simulink library "WECSim_Lib_PTOSim"  (R2020b)
settings: Solver=ode45  StartTime=0.0  StopTime=10.0  RelTol=1e-3  EnableMultiTasking=on
undefined symbols (not defined in the file or in its folder): DiscIntNeverNeededParam, magnitude, ptoSim, simu
libraries: $bdroot x3, simulink x2
(part 2 of 2)

== system WECSim_Lib_PTOSim/Hydraulic/Compressible Fluid Piston/dPa_dt ==
  Pos : Inport
  Vel : Inport  Port=2
  QA : Inport  Port=3
  Add : Sum
  Add1 : Sum  Inputs=+-
  Constant : Constant  Value=ptoSim.hydPistonCompressible.Ap_A
  Constant1 : Constant  Value=ptoSim.hydPistonCompressible.bulkModulus
  Constant2 : Constant  Value=ptoSim.hydPistonCompressible.xi_piston
  Constant3 : Constant  Value=ptoSim.hydPistonCompressible.Ap_A
  Divide : Product  Inputs=/*
  Divide1 : Product  Inputs=*/
  Product : Product
  Product1 : Product
  Saturation : Saturate  UpperLimit=inf  LowerLimit=1e-10
  dPA_dt : Outport
  wires:
  Divide1/1 -> Product1/1
  Constant3/1 -> Divide1/2
  Constant1/1 -> Divide1/1
  Saturation/1 -> Divide/1
  Vel/1 -> Product/1
  Product1/1 -> Divide/2
  Divide/1 -> dPA_dt/1
  Add/1 -> Product1/2
  Constant/1 -> Product/2
  QA/1 -> Add/2
  Product/1 -> Add/1
  Pos/1 -> Add1/2
  Constant2/1 -> Add1/1
  Add1/1 -> Saturation/1

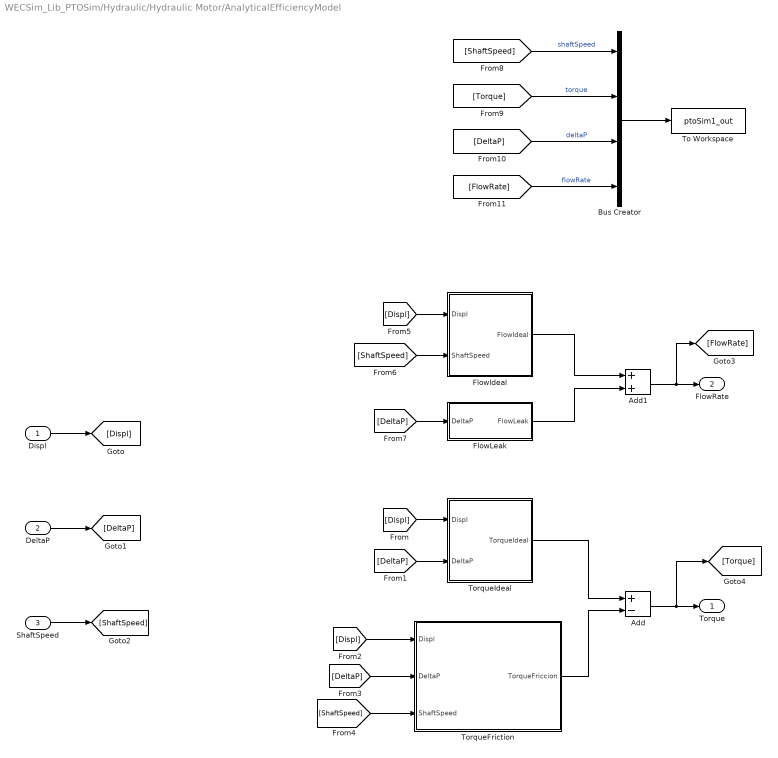
== system WECSim_Lib_PTOSim/Hydraulic/Hydraulic Motor/AnalyticalEfficiencyModel ==
  Displ : Inport
  DeltaP : Inport  Port=2
  ShaftSpeed : Inport  Port=3
  Add : Sum  Inputs=+-
  Add1 : Sum
  Bus Creator : BusCreator  Inputs=4
  FlowIdeal : Subsystem
  FlowLeak : Subsystem
  To Workspace : ToWorkspace  VariableName=ptoSim1_out  SaveFormat=Structure With Time  SampleTime=-1
  TorqueFriction : Subsystem
  TorqueIdeal : Subsystem
  Torque : Outport
  FlowRate : Outport  Port=2
  wires:
  Bus Creator/1 -> To Workspace/1
  Add/1 -> [Torque], Torque/1
  TorqueIdeal/1(TorqueIdeal) -> Add/1
  TorqueFriction/1(TorqueFriccion) -> Add/2
  Displ/1 -> [Displ]
  DeltaP/1 -> [DeltaP]
  ShaftSpeed/1 -> [ShaftSpeed]
  [Displ] -> TorqueIdeal/1(Displ)
  [DeltaP] -> TorqueIdeal/2(DeltaP)
  [DeltaP] -> TorqueFriction/2(DeltaP)
  [Displ] -> TorqueFriction/1(Displ)
  [ShaftSpeed] -> TorqueFriction/3(ShaftSpeed)
  FlowIdeal/1(FlowIdeal) -> Add1/1
  FlowLeak/1(FlowLeak) -> Add1/2
  Add1/1 -> [FlowRate], FlowRate/1
  [Displ] -> FlowIdeal/1(Displ)
  [ShaftSpeed] -> FlowIdeal/2(ShaftSpeed)
  [DeltaP] -> FlowLeak/1(DeltaP)
  [ShaftSpeed] -> Bus Creator/1  "shaftSpeed"
  [Torque] -> Bus Creator/2  "torque"
  [DeltaP] -> Bus Creator/3  "deltaP"
  [FlowRate] -> Bus Creator/4  "flowRate"

== system WECSim_Lib_PTOSim/Hydraulic/Hydraulic Motor/TabulatedEfficiency ==
  Displ : Inport
  DeltaP : Inport  Port=2
  ShaftSpeed : Inport  Port=3
  Bus Creator : BusCreator  Inputs=4
  Constant : Constant  Value=ptoSim.hydraulicMotor.displacement
  Constant2 : Constant  Value=ptoSim.hydraulicMotor.displacement
  Divide : Product  Inputs=/*
  Gain : Gain  Gain=1/((100^3)*(2*pi))
  Gain1 : Gain  Gain=1/((100^3)*(2*pi))
  Gain2 : Gain  Gain=2*pi/60
  MechanicalEfficiency : Lookup_n-D  BreakpointsForDimension1=ptoSim.hydraulicMotor.effTableShaftSpeed  BreakpointsForDimension2=ptoSim.hydraulicMotor.effTableDeltaP  Table=ptoSim.hydraulicMotor.effTableMechEff  InternalRulePriority=Speed  RndMeth=Simplest  InputSameDT=on
      settings: InputPortMap=u0,u1
  Product : Product
  Product1 : Product  Inputs=3
  Product2 : Product
  Product4 : Product
  To Workspace : ToWorkspace  VariableName=ptoSim1_out  SaveFormat=Structure With Time  SampleTime=-1
  VolumetricEfficiency : Lookup_n-D  BreakpointsForDimension1=ptoSim.hydraulicMotor.effTableShaftSpeed  BreakpointsForDimension2=ptoSim.hydraulicMotor.effTableDeltaP  Table=ptoSim.hydraulicMotor.effTableVolEff  InternalRulePriority=Speed  RndMeth=Simplest  InputSameDT=on
      settings: InputPortMap=u0,u1
  Torque : Outport
  FlowRate : Outport  Port=2
  wires:
  ShaftSpeed/1 -> MechanicalEfficiency/2, Gain2/1, VolumetricEfficiency/2, Bus Creator/1  "shaftSpeed"
  Divide/1 -> Bus Creator/4, FlowRate/1  "flowRate"
  Product1/1 -> Bus Creator/2, Torque/1  "torque"
  Gain1/1 -> Product/2
  Product/1 -> Divide/2
  Gain/1 -> Product1/1
  VolumetricEfficiency/1 -> Divide/1
  DeltaP/1 -> Product1/2, VolumetricEfficiency/1, MechanicalEfficiency/1, Bus Creator/3  "deltaP"
  MechanicalEfficiency/1 -> Product1/3
  Product2/1 -> Gain1/1
  Bus Creator/1 -> To Workspace/1
  Product4/1 -> Gain/1
  Constant/1 -> Product2/2
  Displ/1 -> Product4/2, Product2/1
  Constant2/1 -> Product4/1
  Gain2/1 -> Product/1

== system WECSim_Lib_PTOSim/Hydraulic/Rectifying Check Valve/Valve1 ==
  DeltaP : Inport
  Av : Subsystem
  Constant : Constant  Value=ptoSim.rectifyingCheckValve.rho
  Divide : Product  Inputs=/*
  Gain : Gain  Gain=ptoSim.rectifyingCheckValve.k1
  Gain1 : Gain  Gain=2
  Gain2 : Gain  Gain=ptoSim.rectifyingCheckValve.Cd
  Product : Product
  Product1 : Product
  Sqrt : Sqrt  SaturateOnIntegerOverflow=on
  Trigonometric Function : Trigonometry  Operator=tanh
  Qcv : Outport
  wires:
  DeltaP/1 -> Gain/1, Gain1/1, Av/1(DeltaP)
  Gain/1 -> Trigonometric Function/1
  Trigonometric Function/1 -> Product/1
  Gain1/1 -> Product/2
  Product/1 -> Divide/2
  Constant/1 -> Divide/1
  Divide/1 -> Sqrt/1
  Sqrt/1 -> Gain2/1
  Gain2/1 -> Product1/1
  Av/1(Av) -> Product1/2
  Product1/1 -> Qcv/1

== system WECSim_Lib_PTOSim/Motion Conversion/Rotary to Linear Adjustable Rod/Angle Calculation for PTO ==
  angPos : Inport
  Add : Sum  Inputs=+-
  Add1 : Sum  Inputs=+-
  Constant1 : Constant  Value=ptoSim.adjustableRod.crank
  Constant2 : Constant  Value=ptoSim.adjustableRod.crank
  Constant3 : Constant  Value=ptoSim.adjustableRod.offset
  Distance btw flap joint & rod joint along x-axis : Subsystem  AncestorBlock=|
      | PTOSim_Lib/Motion Conversion/Rotary to Linear
      | Adjustable Rod/Angular to Linear
      | Velocity/Subsystem/Distance btw flap joint & rod joint
      | along x-axis
  Divide : Product  Inputs=*/
  Divide1 : Product  Inputs=*/
  Product : Product
  Product1 : Product
  Subsystem1 : Subsystem  AncestorBlock=|
      | PTOSim_Lib/Motion Conversion/Rotary to Linear
      | Adjustable Rod/Angular to Linear
      | Velocity/Subsystem
  Subsystem2 : Subsystem  AncestorBlock=|
      | PTOSim_Lib/Motion Conversion/Rotary to Linear
      | Adjustable Rod/Angular to Linear
      | Velocity/Subsystem
  Trigonometric Function : Trigonometry
  Trigonometric Function1 : Trigonometry  Operator=cos
  Cos_gamma : Outport
  Sin_gamma : Outport  Port=2
  wires:
  Trigonometric Function/1 -> Product/1
  Product/1 -> Add/1
  Distance btw flap joint & rod joint along x-axis/1(d) -> Add/2
  Constant2/1 -> Product/2
  Add/1 -> Divide/1
  Subsystem1/1(rodLength) -> Divide/2
  Divide/1 -> Cos_gamma/1
  Subsystem2/1(rodLength) -> Divide1/2
  Trigonometric Function1/1 -> Product1/1
  Constant1/1 -> Product1/2
  Product1/1 -> Add1/1
  Constant3/1 -> Add1/2
  Add1/1 -> Divide1/1
  angPos/1 -> Subsystem1/1(angPos), Subsystem2/1(angPos), Trigonometric Function1/1, Trigonometric Function/1
  Divide1/1 -> Sin_gamma/1

== system WECSim_Lib_PTOSim/Motion Conversion/Rotary to Linear Adjustable Rod/Angular to Linear Position ==
  angPos : Inport
  Add1 : Sum  Inputs=-+
  Add2 : Sum  Inputs=+-
  Add5 : Sum
  Add6 : Sum  Inputs=+-
  Constant1 : Constant  Value=ptoSim.adjustableRod.rodInit
  Constant2 : Constant  Value=ptoSim.adjustableRod.crank
  Constant3 : Constant  Value=ptoSim.adjustableRod.offset
  Constant7 : Constant  Value=ptoSim.adjustableRod.crank
  Distance btw flap joint & rod joint along x-axis : Subsystem
  Math Function1 : Math  Operator=square  SignedPower=on  SaturateOnIntegerOverflow=on
  Math Function6 : Math  Operator=square  SignedPower=on  SaturateOnIntegerOverflow=on
  Product1 : Product  Inputs=**
  Product7 : Product  Inputs=**
  Sqrt2 : Sqrt  SaturateOnIntegerOverflow=on
  Trigonometric Function1 : Trigonometry  Operator=cos
  Trigonometric Function5 : Trigonometry
  linearPos : Outport
  wires:
  angPos/1 -> Trigonometric Function5/1, Trigonometric Function1/1
  Add1/1 -> linearPos/1
  Add2/1 -> Math Function1/1
  Trigonometric Function5/1 -> Product7/2
  Product7/1 -> Add6/2
  Add6/1 -> Math Function6/1
  Math Function6/1 -> Add5/2
  Add5/1 -> Sqrt2/1
  Sqrt2/1 -> Add1/2
  Constant1/1 -> Add1/1
  Constant2/1 -> Product1/1
  Trigonometric Function1/1 -> Product1/2
  Product1/1 -> Add2/1
  Constant3/1 -> Add2/2
  Math Function1/1 -> Add5/1
  Constant7/1 -> Product7/1
  Distance btw flap joint & rod joint along x-axis/1(d) -> Add6/1

== system WECSim_Lib_PTOSim/Motion Conversion/Rotary to Linear Adjustable Rod/Angular to Linear Velocity ==
  angPos : Inport
  angVel : Inport  Port=2
  Add1 : Sum  Inputs=+-
  Add2 : Sum  Inputs=+-
  Add3 : Sum  Inputs=-+
  Constant1 : Constant  Value=ptoSim.adjustableRod.crank
  Constant2 : Constant  Value=ptoSim.adjustableRod.crank
  Constant3 : Constant  Value=ptoSim.adjustableRod.offset
  Constant7 : Constant  Value=ptoSim.adjustableRod.crank
  Distance btw flap joint & rod joint along x-axis : Subsystem
  Divide1 : Product  Inputs=*/
  Product1 : Product  Inputs=**
  Product2 : Product  Inputs=***
  Product3 : Product  Inputs=**
  Product4 : Product  Inputs=***
  Product7 : Product  Inputs=**
  Subsystem : Subsystem
  Trigonometric Function1 : Trigonometry  Operator=cos
  Trigonometric Function2 : Trigonometry  Operator=cos
  Trigonometric Function5 : Trigonometry
  linearVel : Outport
  wires:
  Add2/1 -> Product2/1
  Constant2/1 -> Product1/1
  Trigonometric Function1/1 -> Product1/2
  Product1/1 -> Add2/1
  Constant3/1 -> Add2/2
  Trigonometric Function5/1 -> Product7/2
  Product7/1 -> Add1/1, Product2/2
  Constant7/1 -> Product7/1
  angVel/1 -> Product2/3, Product4/1
  Distance btw flap joint & rod joint along x-axis/1(d) -> Add1/2
  Constant1/1 -> Product3/1
  Trigonometric Function2/1 -> Product3/2
  Product3/1 -> Product4/3
  angPos/1 -> Trigonometric Function5/1, Trigonometric Function2/1, Trigonometric Function1/1, Subsystem/1(angPos)
  Add1/1 -> Product4/2
  Subsystem/1(rodLength) -> Divide1/2
  Product2/1 -> Add3/1
  Product4/1 -> Add3/2
  Add3/1 -> Divide1/1
  Divide1/1 -> linearVel/1

== system WECSim_Lib_PTOSim/Motion Conversion/Rotary to Linear Crank/Angular to Linear Position ==
  angPos : Inport
  Add1 : Sum  Inputs=++-
  Add2 : Sum  Inputs=+-
  Add5 : Sum  Inputs=+-
  Constant1 : Constant  Value=ptoSim.linearCrank.rodLength
  Constant2 : Constant  Value=ptoSim.linearCrank.crank
  Constant3 : Constant  Value=ptoSim.linearCrank.offset
  Constant7 : Constant  Value=ptoSim.linearCrank.crank
  Initial Distance btw flap joint & crank joint along x-axis : Subsystem
  Math Function1 : Math  Operator=square  SignedPower=on  SaturateOnIntegerOverflow=on
  Math Function2 : Math  Operator=square  SignedPower=on  SaturateOnIntegerOverflow=on
  Product1 : Product  Inputs=**
  Product7 : Product  Inputs=**
  Sqrt2 : Sqrt  SaturateOnIntegerOverflow=on
  Trigonometric Function1 : Trigonometry  Operator=cos
  Trigonometric Function5 : Trigonometry
  linearPos : Outport
  wires:
  angPos/1 -> Trigonometric Function1/1, Trigonometric Function5/1
  Add2/1 -> Math Function1/1
  Trigonometric Function5/1 -> Product7/2
  Add5/1 -> Sqrt2/1
  Constant2/1 -> Product1/1
  Trigonometric Function1/1 -> Product1/2
  Product1/1 -> Add2/1
  Constant3/1 -> Add2/2
  Constant7/1 -> Product7/1
  Initial Distance btw flap joint & crank joint along x-axis/1(d) -> Add1/3
  Constant1/1 -> Math Function2/1
  Math Function1/1 -> Add5/2
  Sqrt2/1 -> Add1/2
  Product7/1 -> Add1/1
  Add1/1 -> linearPos/1
  Math Function2/1 -> Add5/1

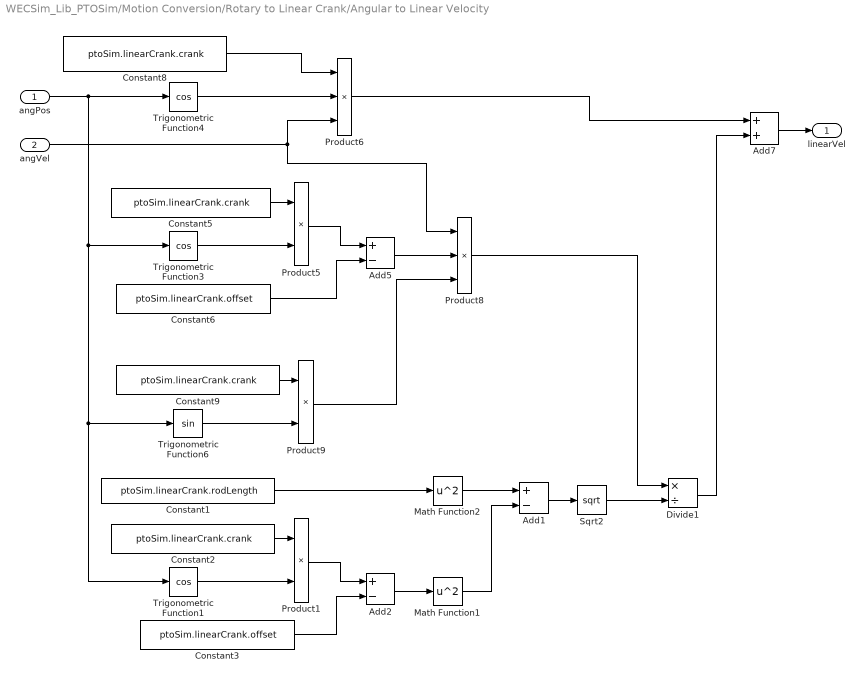
== system WECSim_Lib_PTOSim/Motion Conversion/Rotary to Linear Crank/Angular to Linear Velocity ==
  angPos : Inport
  angVel : Inport  Port=2
  Add1 : Sum  Inputs=+-
  Add2 : Sum  Inputs=+-
  Add5 : Sum  Inputs=+-
  Add7 : Sum
  Constant1 : Constant  Value=ptoSim.linearCrank.rodLength
  Constant{2,5,8..9} (4 alike) : Constant  Value=ptoSim.linearCrank.crank
  Constant3 : Constant  Value=ptoSim.linearCrank.offset
  Constant6 : Constant  Value=ptoSim.linearCrank.offset
  Divide1 : Product  Inputs=*/
  Math Function1 : Math  Operator=square  SignedPower=on  SaturateOnIntegerOverflow=on
  Math Function2 : Math  Operator=square  SignedPower=on  SaturateOnIntegerOverflow=on
  Product1 : Product  Inputs=**
  Product5 : Product  Inputs=**
  Product6 : Product  Inputs=***
  Product8 : Product  Inputs=***
  Product9 : Product  Inputs=**
  Sqrt2 : Sqrt  SaturateOnIntegerOverflow=on
  Trigonometric Function1 : Trigonometry  Operator=cos
  Trigonometric Function3 : Trigonometry  Operator=cos
  Trigonometric Function4 : Trigonometry  Operator=cos
  Trigonometric Function6 : Trigonometry
  linearVel : Outport
  wires:
  Add7/1 -> linearVel/1
  Trigonometric Function4/1 -> Product6/2
  Constant8/1 -> Product6/1
  Product6/1 -> Add7/1
  Constant5/1 -> Product5/1
  Trigonometric Function3/1 -> Product5/2
  Product5/1 -> Add5/1
  Constant6/1 -> Add5/2
  Constant9/1 -> Product9/1
  Trigonometric Function6/1 -> Product9/2
  angVel/1 -> Product8/1, Product6/3
  Add5/1 -> Product8/2
  Product9/1 -> Product8/3
  angPos/1 -> Trigonometric Function1/1, Trigonometric Function6/1, Trigonometric Function3/1, Trigonometric Function4/1
  Add2/1 -> Math Function1/1
  Add1/1 -> Sqrt2/1
  Constant2/1 -> Product1/1
  Trigonometric Function1/1 -> Product1/2
  Product1/1 -> Add2/1
  Constant3/1 -> Add2/2
  Constant1/1 -> Math Function2/1
  Math Function1/1 -> Add1/2
  Sqrt2/1 -> Divide1/2
  Product8/1 -> Divide1/1
  Divide1/1 -> Add7/2
  Math Function2/1 -> Add1/1

== system WECSim_Lib_PTOSim/Motion Conversion/Rotary to Linear Crank/Subsystem ==
  angle : Inport
  Add : Sum  Inputs=+-
  Add1 : Sum  Inputs=+-
  Constant : Constant
  Constant2 : Constant  Value=ptoSim.linearCrank.crank
  Constant3 : Constant  Value=ptoSim.linearCrank.offset
  Constant4 : Constant  Value=ptoSim.linearCrank.rodLength
  Divide : Product  Inputs=*/
  Product : Product
  Sqrt : Sqrt  SaturateOnIntegerOverflow=on
  Square : Math  Operator=square  SignedPower=on  SaturateOnIntegerOverflow=on
  Trigonometric Function : Trigonometry  Operator=cos
  abs(cos_gamma) : Outport
  wires:
  angle/1 -> Trigonometric Function/1
  Trigonometric Function/1 -> Product/1
  Constant2/1 -> Product/2
  Product/1 -> Add/1
  Constant3/1 -> Add/2
  Add/1 -> Divide/1
  Constant4/1 -> Divide/2
  Divide/1 -> Square/1
  Square/1 -> Add1/2
  Add1/1 -> Sqrt/1
  Constant/1 -> Add1/1
  Sqrt/1 -> abs(cos_gamma)/1

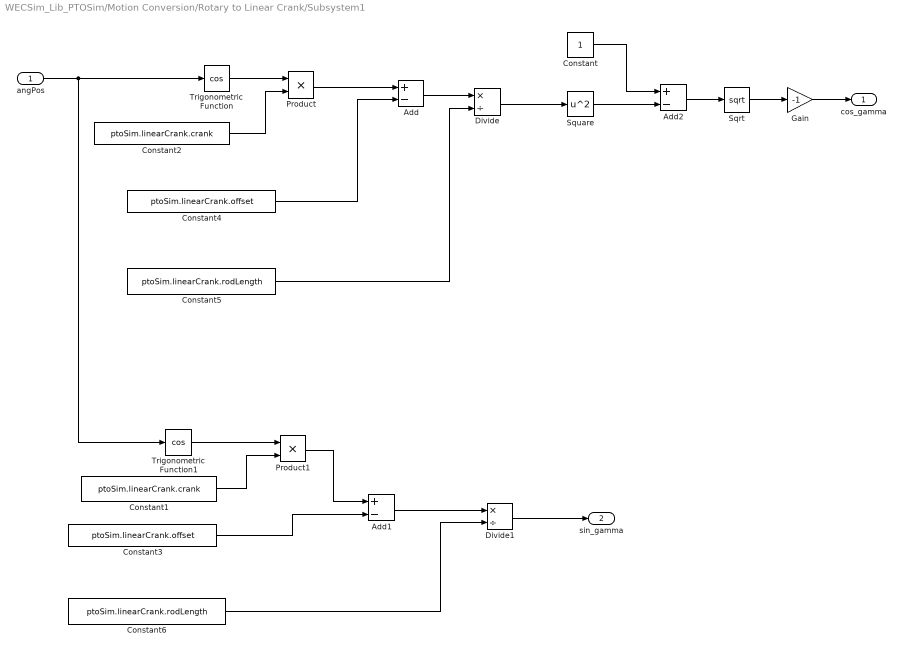
== system WECSim_Lib_PTOSim/Motion Conversion/Rotary to Linear Crank/Subsystem1 ==
  angPos : Inport
  Add : Sum  Inputs=+-
  Add1 : Sum  Inputs=+-
  Add2 : Sum  Inputs=+-
  Constant : Constant
  Constant1 : Constant  Value=ptoSim.linearCrank.crank
  Constant2 : Constant  Value=ptoSim.linearCrank.crank
  Constant3 : Constant  Value=ptoSim.linearCrank.offset
  Constant4 : Constant  Value=ptoSim.linearCrank.offset
  Constant5 : Constant  Value=ptoSim.linearCrank.rodLength
  Constant6 : Constant  Value=ptoSim.linearCrank.rodLength
  Divide : Product  Inputs=*/
  Divide1 : Product  Inputs=*/
  Gain : Gain  Gain=-1
  Product : Product
  Product1 : Product
  Sqrt : Sqrt  SaturateOnIntegerOverflow=on
  Square : Math  Operator=square  SignedPower=on  SaturateOnIntegerOverflow=on
  Trigonometric Function : Trigonometry  Operator=cos
  Trigonometric Function1 : Trigonometry  Operator=cos
  cos_gamma : Outport
  sin_gamma : Outport  Port=2
  wires:
  Divide1/1 -> sin_gamma/1
  Add1/1 -> Divide1/1
  Constant3/1 -> Add1/2
  Product1/1 -> Add1/1
  Constant1/1 -> Product1/2
  Trigonometric Function1/1 -> Product1/1
  Constant6/1 -> Divide1/2
  Add/1 -> Divide/1
  Add2/1 -> Sqrt/1
  angPos/1 -> Trigonometric Function1/1, Trigonometric Function/1
  Square/1 -> Add2/2
  Product/1 -> Add/1
  Constant2/1 -> Product/2
  Trigonometric Function/1 -> Product/1
  Divide/1 -> Square/1
  Constant5/1 -> Divide/2
  Constant/1 -> Add2/1
  Constant4/1 -> Add/2
  Sqrt/1 -> Gain/1
  Gain/1 -> cos_gamma/1

== system WECSim_Lib_PTOSim/Hydraulic/Hydraulic Motor/AnalyticalEfficiencyModel/FlowIdeal ==
  Displ : Inport
  ShaftSpeed : Inport  Port=2
  Constant1 : Constant  Value=ptoSim.hydraulicMotor.displacement
  Gain : Gain  Gain=1/((100^3)*60)
  Product : Product  Inputs=3
  FlowIdeal : Outport
  wires:
  Constant1/1 -> Product/1
  Displ/1 -> Product/2
  ShaftSpeed/1 -> Product/3
  Product/1 -> Gain/1
  Gain/1 -> FlowIdeal/1

== system WECSim_Lib_PTOSim/Hydraulic/Hydraulic Motor/AnalyticalEfficiencyModel/FlowLeak ==
  DeltaP : Inport
  Add : Sum  Inputs=+-
  Constant : Constant
  Constant1 : Constant  Value=ptoSim.hydraulicMotor.visNominal
  Constant2 : Constant  Value=ptoSim.hydraulicMotor.densityNominal
  Constant3 : Constant  Value=ptoSim.hydraulicMotor.wNominal
  Constant4 : Constant  Value=ptoSim.hydraulicMotor.displacement
  Constant5 : Constant
  Constant6 : Constant  Value=ptoSim.hydraulicMotor.effVolNom
  Constant7 : Constant  Value=ptoSim.hydraulicMotor.rho
  Constant8 : Constant  Value=ptoSim.hydraulicMotor.viscosity
  Constant9 : Constant  Value=ptoSim.hydraulicMotor.deltaPNominal
  Divide : Product  Inputs=*/
  Divide1 : Product  Inputs=*/
  Gain : Gain  Gain=2*pi/60
  Gain1 : Gain  Gain=1/((100^3)*(2*pi))
  Product : Product
  Product1 : Product  Inputs=5
  Product2 : Product  Inputs=3
  FlowLeak : Outport
  wires:
  DeltaP/1 -> Product/1
  Constant1/1 -> Product1/1
  Constant2/1 -> Product1/2
  Constant3/1 -> Gain/1
  Gain/1 -> Product1/3
  Constant4/1 -> Gain1/1
  Gain1/1 -> Product1/4
  Add/1 -> Product1/5
  Constant/1 -> Add/2
  Divide/1 -> Add/1
  Constant5/1 -> Divide/1
  Constant6/1 -> Divide/2
  Product/1 -> FlowLeak/1
  Product1/1 -> Divide1/1
  Product2/1 -> Divide1/2
  Divide1/1 -> Product/2
  Constant7/1 -> Product2/1
  Constant8/1 -> Product2/2
  Constant9/1 -> Product2/3

== system WECSim_Lib_PTOSim/Hydraulic/Hydraulic Motor/AnalyticalEfficiencyModel/TorqueFriction ==
  Displ : Inport
  DeltaP : Inport  Port=2
  ShaftSpeed : Inport  Port=3
  Abs : Abs
  Abs1 : Abs
  Add : Sum
  Constant : Constant  Value=ptoSim.hydraulicMotor.torqueNoLoad
  Constant1 : Constant  Value=ptoSim.hydraulicMotor.torqueVsPressure
  Constant3 : Constant  Value=ptoSim.hydraulicMotor.wNominal
  Divide1 : Product  Inputs=*/
  Gain : Gain  Gain=4
  Gain1 : Gain  Gain=0.01
  Product : Product  Inputs=3
  Product1 : Product
  Tanh : Trigonometry  Operator=tanh
  TorqueFriccion : Outport
  wires:
  Constant/1 -> Add/1
  Product/1 -> Add/2
  Constant1/1 -> Product/1
  Displ/1 -> Abs/1
  Abs/1 -> Product/2
  DeltaP/1 -> Abs1/1
  Abs1/1 -> Product/3
  Add/1 -> Product1/2
  ShaftSpeed/1 -> Gain/1
  Constant3/1 -> Gain1/1
  Gain/1 -> Divide1/1
  Gain1/1 -> Divide1/2
  Divide1/1 -> Tanh/1
  Tanh/1 -> Product1/1
  Product1/1 -> TorqueFriccion/1

== system WECSim_Lib_PTOSim/Hydraulic/Hydraulic Motor/AnalyticalEfficiencyModel/TorqueIdeal ==
  Displ : Inport
  DeltaP : Inport  Port=2
  Constant1 : Constant  Value=ptoSim.hydraulicMotor.displacement
  Gain : Gain  Gain=1/((100^3)*(2*pi))
  Product : Product
  Product1 : Product
  TorqueIdeal : Outport
  wires:
  Product/1 -> TorqueIdeal/1
  Gain/1 -> Product/1
  DeltaP/1 -> Product/2
  Product1/1 -> Gain/1
  Displ/1 -> Product1/2
  Constant1/1 -> Product1/1

== system WECSim_Lib_PTOSim/Hydraulic/Rectifying Check Valve/Valve1/Av ==
  DeltaP : Inport
  Add : Sum
  Add1 : Sum  Inputs=+-
  Add2 : Sum  Inputs=+-
  Add3 : Sum
  Add4 : Sum
  Constant : Constant
  Constant1 : Constant  Value=ptoSim.rectifyingCheckValve.Amax
  Constant2 : Constant  Value=ptoSim.rectifyingCheckValve.Amin
  Constant3 : Constant  Value=ptoSim.rectifyingCheckValve.pMax
  Constant4 : Constant  Value=ptoSim.rectifyingCheckValve.pMin
  Constant5 : Constant  Value=ptoSim.rectifyingCheckValve.Amin
  Gain : Gain  Gain=ptoSim.rectifyingCheckValve.k2
  Gain1 : Gain  Gain=0.5
  Gain2 : Gain  Gain=0.5
  Product : Product
  Trigonometric Function : Trigonometry  Operator=tanh
  Av : Outport
  wires:
  Constant5/1 -> Add4/1
  Product/1 -> Add4/2
  Constant3/1 -> Add3/1
  Gain/1 -> Trigonometric Function/1
  Add2/1 -> Gain/1
  Constant/1 -> Add/2
  Add1/1 -> Gain2/1
  Constant1/1 -> Add1/1
  Trigonometric Function/1 -> Add/1
  Add3/1 -> Gain1/1
  Constant2/1 -> Add1/2
  Gain1/1 -> Add2/2
  Constant4/1 -> Add3/2
  Add/1 -> Product/1
  Gain2/1 -> Product/2
  Add4/1 -> Av/1
  DeltaP/1 -> Add2/1

== system WECSim_Lib_PTOSim/Motion Conversion/Rotary to Linear Adjustable Rod/Angle Calculation for PTO/Distance btw flap joint & rod joint along x-axis ==
  Add3 : Sum  Inputs=+-
  Add4 : Sum  Inputs=+-
  Constant4 : Constant  Value=ptoSim.adjustableRod.rodInit
  Constant5 : Constant  Value=ptoSim.adjustableRod.crank
  Constant6 : Constant  Value=ptoSim.adjustableRod.offset
  Math Function2 : Math  Operator=square  SignedPower=on  SaturateOnIntegerOverflow=on
  Math Function3 : Math  Operator=square  SignedPower=on  SaturateOnIntegerOverflow=on
  Sqrt1 : Sqrt  SaturateOnIntegerOverflow=on
  d : Outport
  wires:
  Sqrt1/1 -> d/1
  Math Function2/1 -> Add3/1
  Math Function3/1 -> Add3/2
  Add4/1 -> Math Function3/1
  Constant6/1 -> Add4/2
  Constant5/1 -> Add4/1
  Constant4/1 -> Math Function2/1
  Add3/1 -> Sqrt1/1

== system WECSim_Lib_PTOSim/Motion Conversion/Rotary to Linear Adjustable Rod/Angle Calculation for PTO/Subsystem1 ==
  angPos : Inport
  Add2 : Sum  Inputs=+-
  Add5 : Sum
  Add6 : Sum  Inputs=+-
  Constant1 : Constant  Value=ptoSim.adjustableRod.crank
  Constant2 : Constant  Value=ptoSim.adjustableRod.crank
  Constant3 : Constant  Value=ptoSim.adjustableRod.offset
  Distance btw flap joint & rod joint along x-axis : Subsystem
  Math Function1 : Math  Operator=square  SignedPower=on  SaturateOnIntegerOverflow=on
  Math Function6 : Math  Operator=square  SignedPower=on  SaturateOnIntegerOverflow=on
  Product1 : Product  Inputs=**
  Product7 : Product  Inputs=**
  Sqrt2 : Sqrt  SaturateOnIntegerOverflow=on
  Trigonometric Function1 : Trigonometry  Operator=cos
  Trigonometric Function5 : Trigonometry
  rodLength : Outport
  wires:
  Distance btw flap joint & rod joint along x-axis/1(d) -> Add6/1
  Constant2/1 -> Product7/1
  Math Function1/1 -> Add5/1
  Constant3/1 -> Add2/2
  Product1/1 -> Add2/1
  Trigonometric Function1/1 -> Product1/2
  Constant1/1 -> Product1/1
  Sqrt2/1 -> rodLength/1
  Add5/1 -> Sqrt2/1
  Math Function6/1 -> Add5/2
  Add6/1 -> Math Function6/1
  Product7/1 -> Add6/2
  Trigonometric Function5/1 -> Product7/2
  Add2/1 -> Math Function1/1
  angPos/1 -> Trigonometric Function1/1, Trigonometric Function5/1

== system WECSim_Lib_PTOSim/Motion Conversion/Rotary to Linear Adjustable Rod/Angle Calculation for PTO/Subsystem2 ==
  angPos : Inport
  Add2 : Sum  Inputs=+-
  Add5 : Sum
  Add6 : Sum  Inputs=+-
  Constant1 : Constant  Value=ptoSim.adjustableRod.crank
  Constant2 : Constant  Value=ptoSim.adjustableRod.crank
  Constant3 : Constant  Value=ptoSim.adjustableRod.offset
  Distance btw flap joint & rod joint along x-axis : Subsystem
  Math Function1 : Math  Operator=square  SignedPower=on  SaturateOnIntegerOverflow=on
  Math Function6 : Math  Operator=square  SignedPower=on  SaturateOnIntegerOverflow=on
  Product1 : Product  Inputs=**
  Product7 : Product  Inputs=**
  Sqrt2 : Sqrt  SaturateOnIntegerOverflow=on
  Trigonometric Function1 : Trigonometry  Operator=cos
  Trigonometric Function5 : Trigonometry
  rodLength : Outport
  wires:
  Distance btw flap joint & rod joint along x-axis/1(d) -> Add6/1
  Constant2/1 -> Product7/1
  Math Function1/1 -> Add5/1
  Constant3/1 -> Add2/2
  Product1/1 -> Add2/1
  Trigonometric Function1/1 -> Product1/2
  Constant1/1 -> Product1/1
  Sqrt2/1 -> rodLength/1
  Add5/1 -> Sqrt2/1
  Math Function6/1 -> Add5/2
  Add6/1 -> Math Function6/1
  Product7/1 -> Add6/2
  Trigonometric Function5/1 -> Product7/2
  Add2/1 -> Math Function1/1
  angPos/1 -> Trigonometric Function1/1, Trigonometric Function5/1

== system WECSim_Lib_PTOSim/Motion Conversion/Rotary to Linear Adjustable Rod/Angular to Linear Position/Distance btw flap joint & rod joint along x-axis ==
  Add3 : Sum  Inputs=+-
  Add4 : Sum  Inputs=+-
  Constant4 : Constant  Value=ptoSim.adjustableRod.rodInit
  Constant5 : Constant  Value=ptoSim.adjustableRod.crank
  Constant6 : Constant  Value=ptoSim.adjustableRod.offset
  Math Function2 : Math  Operator=square  SignedPower=on  SaturateOnIntegerOverflow=on
  Math Function3 : Math  Operator=square  SignedPower=on  SaturateOnIntegerOverflow=on
  Sqrt1 : Sqrt  SaturateOnIntegerOverflow=on
  d : Outport
  wires:
  Add3/1 -> Sqrt1/1
  Constant4/1 -> Math Function2/1
  Constant5/1 -> Add4/1
  Constant6/1 -> Add4/2
  Add4/1 -> Math Function3/1
  Math Function3/1 -> Add3/2
  Math Function2/1 -> Add3/1
  Sqrt1/1 -> d/1

== system WECSim_Lib_PTOSim/Motion Conversion/Rotary to Linear Adjustable Rod/Angular to Linear Velocity/Distance btw flap joint & rod joint along x-axis ==
  Add3 : Sum  Inputs=+-
  Add4 : Sum  Inputs=+-
  Constant4 : Constant  Value=ptoSim.adjustableRod.rodInit
  Constant5 : Constant  Value=ptoSim.adjustableRod.crank
  Constant6 : Constant  Value=ptoSim.adjustableRod.offset
  Math Function2 : Math  Operator=square  SignedPower=on  SaturateOnIntegerOverflow=on
  Math Function3 : Math  Operator=square  SignedPower=on  SaturateOnIntegerOverflow=on
  Sqrt1 : Sqrt  SaturateOnIntegerOverflow=on
  d : Outport
  wires:
  Add3/1 -> Sqrt1/1
  Constant4/1 -> Math Function2/1
  Constant5/1 -> Add4/1
  Constant6/1 -> Add4/2
  Add4/1 -> Math Function3/1
  Math Function3/1 -> Add3/2
  Math Function2/1 -> Add3/1
  Sqrt1/1 -> d/1

== system WECSim_Lib_PTOSim/Motion Conversion/Rotary to Linear Adjustable Rod/Angular to Linear Velocity/Subsystem ==
  angPos : Inport
  Add2 : Sum  Inputs=+-
  Add5 : Sum
  Add6 : Sum  Inputs=+-
  Constant2 : Constant  Value=ptoSim.adjustableRod.crank
  Constant3 : Constant  Value=ptoSim.adjustableRod.offset
  Constant7 : Constant  Value=ptoSim.adjustableRod.crank
  Distance btw flap joint & rod joint along x-axis : Subsystem
  Math Function1 : Math  Operator=square  SignedPower=on  SaturateOnIntegerOverflow=on
  Math Function6 : Math  Operator=square  SignedPower=on  SaturateOnIntegerOverflow=on
  Product1 : Product  Inputs=**
  Product7 : Product  Inputs=**
  Sqrt2 : Sqrt  SaturateOnIntegerOverflow=on
  Trigonometric Function1 : Trigonometry  Operator=cos
  Trigonometric Function5 : Trigonometry
  rodLength : Outport
  wires:
  angPos/1 -> Trigonometric Function5/1, Trigonometric Function1/1
  Add2/1 -> Math Function1/1
  Trigonometric Function5/1 -> Product7/2
  Product7/1 -> Add6/2
  Add6/1 -> Math Function6/1
  Math Function6/1 -> Add5/2
  Add5/1 -> Sqrt2/1
  Sqrt2/1 -> rodLength/1
  Constant2/1 -> Product1/1
  Trigonometric Function1/1 -> Product1/2
  Product1/1 -> Add2/1
  Constant3/1 -> Add2/2
  Math Function1/1 -> Add5/1
  Constant7/1 -> Product7/1
  Distance btw flap joint & rod joint along x-axis/1(d) -> Add6/1

== system WECSim_Lib_PTOSim/Motion Conversion/Rotary to Linear Crank/Angular to Linear Position/Initial Distance btw flap joint & crank joint along x-axis ==
  Add3 : Sum  Inputs=+-
  Add4 : Sum  Inputs=+-
  Constant1 : Constant  Value=ptoSim.linearCrank.rodLength
  Constant5 : Constant  Value=ptoSim.linearCrank.crank
  Constant6 : Constant  Value=ptoSim.linearCrank.offset
  Math Function2 : Math  Operator=square  SignedPower=on  SaturateOnIntegerOverflow=on
  Math Function3 : Math  Operator=square  SignedPower=on  SaturateOnIntegerOverflow=on
  Sqrt1 : Sqrt  SaturateOnIntegerOverflow=on
  d : Outport
  wires:
  Add3/1 -> Sqrt1/1
  Constant1/1 -> Math Function2/1
  Constant5/1 -> Add4/1
  Constant6/1 -> Add4/2
  Add4/1 -> Math Function3/1
  Math Function3/1 -> Add3/2
  Math Function2/1 -> Add3/1
  Sqrt1/1 -> d/1

== system WECSim_Lib_PTOSim/Motion Conversion/Rotary to Linear Adjustable Rod/Angle Calculation for PTO/Subsystem1/Distance btw flap joint & rod joint along x-axis ==
  Add3 : Sum  Inputs=+-
  Add4 : Sum  Inputs=+-
  Constant1 : Constant  Value=ptoSim.adjustableRod.crank
  Constant2 : Constant  Value=ptoSim.adjustableRod.rodInit
  Constant3 : Constant  Value=ptoSim.adjustableRod.offset
  Math Function2 : Math  Operator=square  SignedPower=on  SaturateOnIntegerOverflow=on
  Math Function3 : Math  Operator=square  SignedPower=on  SaturateOnIntegerOverflow=on
  Sqrt1 : Sqrt  SaturateOnIntegerOverflow=on
  d : Outport
  wires:
  Sqrt1/1 -> d/1
  Math Function2/1 -> Add3/1
  Math Function3/1 -> Add3/2
  Add4/1 -> Math Function3/1
  Constant3/1 -> Add4/2
  Constant1/1 -> Add4/1
  Constant2/1 -> Math Function2/1
  Add3/1 -> Sqrt1/1

== system WECSim_Lib_PTOSim/Motion Conversion/Rotary to Linear Adjustable Rod/Angle Calculation for PTO/Subsystem2/Distance btw flap joint & rod joint along x-axis ==
  Add3 : Sum  Inputs=+-
  Add4 : Sum  Inputs=+-
  Constant1 : Constant  Value=ptoSim.adjustableRod.crank
  Constant2 : Constant  Value=ptoSim.adjustableRod.rodInit
  Constant3 : Constant  Value=ptoSim.adjustableRod.offset
  Math Function2 : Math  Operator=square  SignedPower=on  SaturateOnIntegerOverflow=on
  Math Function3 : Math  Operator=square  SignedPower=on  SaturateOnIntegerOverflow=on
  Sqrt1 : Sqrt  SaturateOnIntegerOverflow=on
  d : Outport
  wires:
  Sqrt1/1 -> d/1
  Math Function2/1 -> Add3/1
  Math Function3/1 -> Add3/2
  Add4/1 -> Math Function3/1
  Constant3/1 -> Add4/2
  Constant1/1 -> Add4/1
  Constant2/1 -> Math Function2/1
  Add3/1 -> Sqrt1/1

== system WECSim_Lib_PTOSim/Motion Conversion/Rotary to Linear Adjustable Rod/Angular to Linear Velocity/Subsystem/Distance btw flap joint & rod joint along x-axis ==
  Add3 : Sum  Inputs=+-
  Add4 : Sum  Inputs=+-
  Constant4 : Constant  Value=ptoSim.adjustableRod.rodInit
  Constant5 : Constant  Value=ptoSim.adjustableRod.crank
  Constant6 : Constant  Value=ptoSim.adjustableRod.offset
  Math Function2 : Math  Operator=square  SignedPower=on  SaturateOnIntegerOverflow=on
  Math Function3 : Math  Operator=square  SignedPower=on  SaturateOnIntegerOverflow=on
  Sqrt1 : Sqrt  SaturateOnIntegerOverflow=on
  d : Outport
  wires:
  Add3/1 -> Sqrt1/1
  Constant4/1 -> Math Function2/1
  Constant5/1 -> Add4/1
  Constant6/1 -> Add4/2
  Add4/1 -> Math Function3/1
  Math Function3/1 -> Add3/2
  Math Function2/1 -> Add3/1
  Sqrt1/1 -> d/1
